simulink model "DIY_simuling"  (R2019a)
settings: Solver=ode23t  StartTime=0.0  StopTime=10  MaxStep=0.2  RelTol=1e-3
model workspace: external: MATLAB File D:\Users\bahaa\Desktop\gra_project\MATLAB\Assem1_DataFile.m (data not in the file)
undefined symbols (not defined in the file): ARM, J2, J3, J4, LEFT, RIGHT, Robot, smiData, TOP, X, Y, Z
libraries: sm_lib x92, nesl_utility x19
(part 1 of 3)
settings Model: Creator=bahaa  LastModifiedBy=bahaa

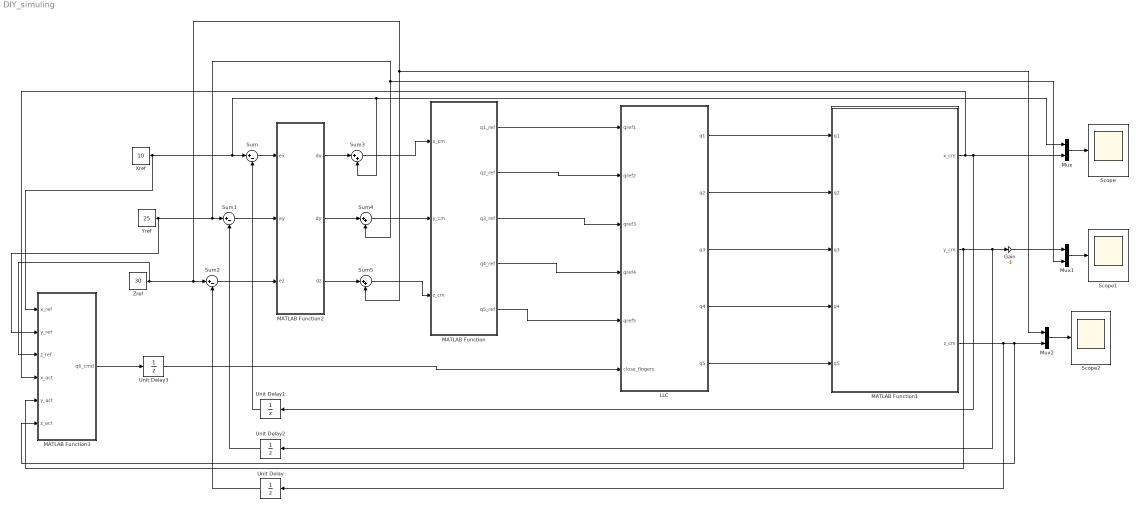
== system DIY_simuling ==
  Gain : Gain  Gain=-1
  LLC : Subsystem
  MATLAB Function : MATLAB Function  TreatAsAtomicUnit=on
  MATLAB Function1 : MATLAB Function  TreatAsAtomicUnit=on
  MATLAB Function2 : MATLAB Function  TreatAsAtomicUnit=on
  MATLAB Function3 : MATLAB Function  TreatAsAtomicUnit=on
  Mux : Mux  Inputs=2
  Mux1 : Mux  Inputs=2
  Mux2 : Mux  Inputs=2
  Scope : Scope
  Scope1 : Scope
  Scope2 : Scope
  Sum : Sum  Inputs=|+-
  Sum1 : Sum  Inputs=|+-
  Sum2 : Sum  Inputs=|+-
  Sum3 : Sum  Inputs=|++
  Sum4 : Sum  Inputs=|++
  Sum5 : Sum  Inputs=|++
  Unit Delay{,1..3} (4 alike) : UnitDelay  SampleTime=-1  HasFrameUpgradeWarning=on
  Xref : Constant  Value=10
  Yref : Constant  Value=25
  Zref : Constant  Value=30
  wires:
  Xref/1 -> MATLAB Function3/1(x_ref), Mux/1, Sum3/2, Sum/1
  Zref/1 -> MATLAB Function3/3(z_ref), Sum2/1, Sum5/2, Mux2/1
  Sum/1 -> MATLAB Function2/1(ex)
  Sum1/1 -> MATLAB Function2/2(ey)
  Sum2/1 -> MATLAB Function2/3(ez)
  MATLAB Function/1(q1_ref) -> LLC/1(qref1)
  MATLAB Function/2(q2_ref) -> LLC/2(qref2)
  MATLAB Function/3(q3_ref) -> LLC/3(qref3)
  MATLAB Function/4(q4_ref) -> LLC/4(qref4)
  MATLAB Function/5(q5_ref) -> LLC/5(qref5)
  LLC/1(q1) -> MATLAB Function1/1(q1)
  LLC/2(q2) -> MATLAB Function1/2(q2)
  LLC/3(q3) -> MATLAB Function1/3(q3)
  LLC/4(q4) -> MATLAB Function1/4(q4)
  LLC/5(q5) -> MATLAB Function1/5(q5)
  MATLAB Function1/2(y_cm) -> MATLAB Function3/5(y_act), Unit Delay2/1, Gain/1
  MATLAB Function1/3(z_cm) -> MATLAB Function3/6(z_act), Mux2/2, Unit Delay/1
  Mux/1 -> Scope/1
  Mux1/1 -> Scope1/1
  Mux2/1 -> Scope2/1
  MATLAB Function2/1(dx) -> Sum3/1
  MATLAB Function2/2(dy) -> Sum4/1
  MATLAB Function2/3(dz) -> Sum5/1
  Sum3/1 -> MATLAB Function/1(x_cm)
  Sum4/1 -> MATLAB Function/2(y_cm)
  Sum5/1 -> MATLAB Function/3(z_cm)
  Unit Delay/1 -> Sum2/2
  Unit Delay1/1 -> Sum/2
  Unit Delay2/1 -> Sum1/2
  MATLAB Function1/1(x_cm) -> MATLAB Function3/4(x_act), Mux/2, Unit Delay1/1
  MATLAB Function3/1(q6_cmd) -> Unit Delay3/1
  Unit Delay3/1 -> LLC/6(close_fingers)
  Yref/1 -> MATLAB Function3/2(y_ref), Mux1/2, Sum4/2, Sum1/1
  Gain/1 -> Mux1/1

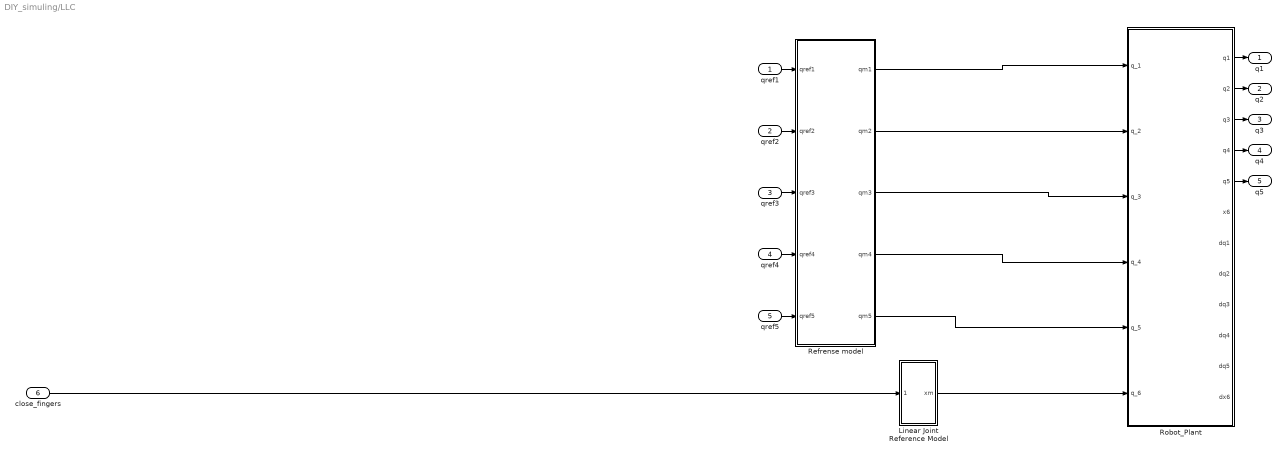
== system DIY_simuling/LLC ==
  qref1 : Inport
  qref2 : Inport  Port=2
  qref3 : Inport  Port=3
  qref4 : Inport  Port=4
  qref5 : Inport  Port=5
  close_fingers : Inport  Port=6
  Linear Joint Reference Model : Subsystem
  Refrense model : Subsystem
  Robot_Plant : Subsystem
  q1 : Outport
  q2 : Outport  Port=2
  q3 : Outport  Port=3
  q4 : Outport  Port=4
  q5 : Outport  Port=5
  wires:
  qref1/1 -> Refrense model/1(qref1)
  Refrense model/4(qm4) -> Robot_Plant/4(q_4)
  Refrense model/3(qm3) -> Robot_Plant/3(q_3)
  Linear Joint Reference Model/1(xm) -> Robot_Plant/6(q_6)
  Refrense model/1(qm1) -> Robot_Plant/1(q_1)
  Refrense model/2(qm2) -> Robot_Plant/2(q_2)
  Refrense model/5(qm5) -> Robot_Plant/5(q_5)
  Robot_Plant/1(q1) -> q1/1
  qref2/1 -> Refrense model/2(qref2)
  qref4/1 -> Refrense model/4(qref4)
  qref3/1 -> Refrense model/3(qref3)
  qref5/1 -> Refrense model/5(qref5)
  Robot_Plant/4(q4) -> q4/1
  Robot_Plant/3(q3) -> q3/1
  Robot_Plant/2(q2) -> q2/1
  Robot_Plant/5(q5) -> q5/1
  close_fingers/1 -> Linear Joint Reference Model/1(x6ref)

== system DIY_simuling/LLC/Linear Joint Reference Model ==
  x6ref : Inport
  Integrator : Integrator  InitialCondition=[0;0]
  MATLAB Function : MATLAB Function  TreatAsAtomicUnit=on
  xm : Outport
  wires:
  Integrator/1 -> MATLAB Function/2(xm6)
  MATLAB Function/1(xm6dot) -> Integrator/1
  MATLAB Function/2(x6_m) -> xm/1
  x6ref/1 -> MATLAB Function/1(x6_ref)

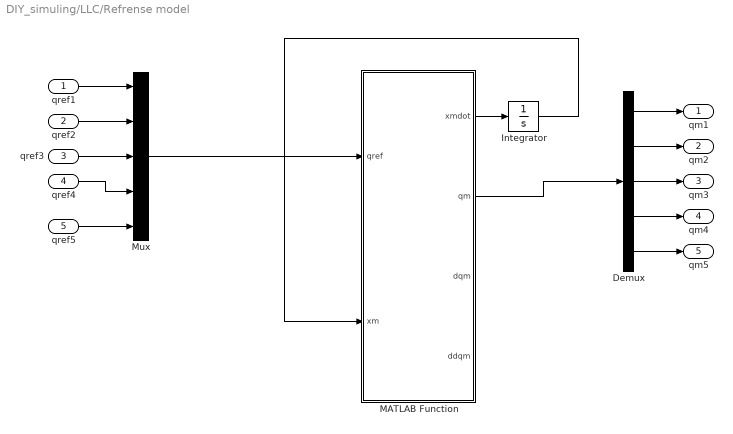
== system DIY_simuling/LLC/Refrense model ==
  qref1 : Inport
  qref2 : Inport  Port=2
  qref3 : Inport  Port=3
  qref4 : Inport  Port=4
  qref5 : Inport  Port=5
  Demux : Demux  Outputs=5
  Integrator : Integrator  InitialCondition=zeros(10,1)
  MATLAB Function : MATLAB Function  TreatAsAtomicUnit=on
  Mux : Mux  Inputs=5
  qm1 : Outport
  qm2 : Outport  Port=2
  qm3 : Outport  Port=3
  qm4 : Outport  Port=4
  qm5 : Outport  Port=5
  wires:
  MATLAB Function/1(xmdot) -> Integrator/1
  MATLAB Function/2(qm) -> Demux/1
  Integrator/1 -> MATLAB Function/2(xm)
  Demux/5 -> qm5/1
  Demux/4 -> qm4/1
  Demux/3 -> qm3/1
  Demux/2 -> qm2/1
  Demux/1 -> qm1/1
  qref1/1 -> Mux/1
  Mux/1 -> MATLAB Function/1(qref)
  qref2/1 -> Mux/2
  qref3/1 -> Mux/3
  qref4/1 -> Mux/4
  qref5/1 -> Mux/5

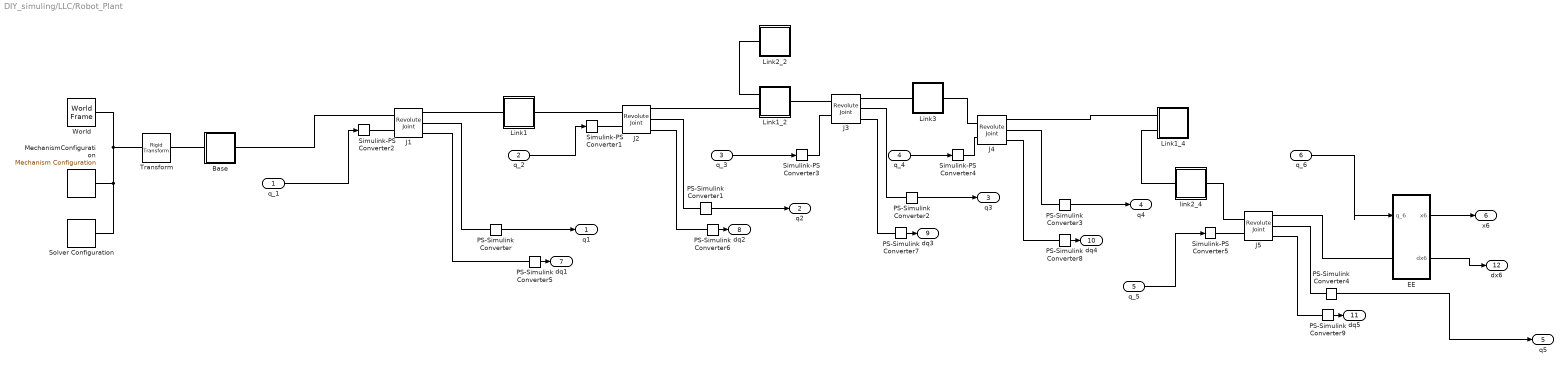
== system DIY_simuling/LLC/Robot_Plant ==
  q_1 : Inport
  q_2 : Inport  Port=2
  q_3 : Inport  Port=3
  q_4 : Inport  Port=4
  q_5 : Inport  Port=5
  q_6 : Inport  Port=6
  Base : Subsystem
  EE : Subsystem
  J1 : sm_lib/Joints/Revolute Joint  SenseConstraintForce=off  SenseConstraintForceX=off  SenseConstraintForceY=off  SenseConstraintForceZ=off  SenseConstraintTorque=off  SenseConstraintTorqueX=off  SenseConstraintTorqueY=off  SenseConstraintTorqueZ=off  SenseTotalForce=off  SenseTotalForceX=off  SenseTotalForceY=off  SenseTotalForceZ=off  SenseTotalTorque=off  SenseTotalTorqueX=off  SenseTotalTorqueY=off  SenseTotalTorqueZ=off  CompositeWrenchDir=FollowerOnBase  CompositeWrenchFrame=BaseFrame  EquilibriumPosition=0  EquilibriumPositionUnits=rad  SpringStiffness=0  SpringStiffnessUnits=N*m/rad  DampingCoefficient=0  DampingCoefficientUnits=N*m/(rad/s)  TorqueActuationMode=ComputedTorque  MotionActuationMode=InputMotion  SensePosition=on  SenseVelocity=on  SenseAcceleration=off  SenseTorqueForce=off  SenseLowerLimitTorqueForce=off  SenseUpperLimitTorqueForce=off  LowerLimitSpecify=on  LowerLimitBound=-90  LowerLimitBoundUnits=deg  LowerLimitStiffness=1e4  LowerLimitStiffnessUnits=N*m/deg  LowerLimitDamping=10  LowerLimitDampingUnits=N*m/(deg/s)  LowerLimitTransitionRegionWidth=0.1  LowerLimitTransitionRegionWidthUnits=deg  UpperLimitSpecify=on  UpperLimitBound=90  UpperLimitBoundUnits=deg  UpperLimitStiffness=1e4  UpperLimitStiffnessUnits=N*m/deg  UpperLimitDamping=10  UpperLimitDampingUnits=N*m/(deg/s)  UpperLimitTransitionRegionWidth=0.1  UpperLimitTransitionRegionWidthUnits=deg  PositionTargetSpecify=on  PositionTargetPriority=Low  PositionTargetValue=smiData.RevoluteJoint(5).Rz.Pos  PositionTargetValueUnits=deg  VelocityTargetSpecify=off  VelocityTargetPriority=High  VelocityTargetValue=0  VelocityTargetValueUnits=deg/s
  J2 : sm_lib/Joints/Revolute Joint  SenseConstraintForce=off  SenseConstraintForceX=off  SenseConstraintForceY=off  SenseConstraintForceZ=off  SenseConstraintTorque=off  SenseConstraintTorqueX=off  SenseConstraintTorqueY=off  SenseConstraintTorqueZ=off  SenseTotalForce=off  SenseTotalForceX=off  SenseTotalForceY=off  SenseTotalForceZ=off  SenseTotalTorque=off  SenseTotalTorqueX=off  SenseTotalTorqueY=off  SenseTotalTorqueZ=off  CompositeWrenchDir=FollowerOnBase  CompositeWrenchFrame=BaseFrame  EquilibriumPosition=0  EquilibriumPositionUnits=rad  SpringStiffness=0  SpringStiffnessUnits=N*m/rad  DampingCoefficient=0  DampingCoefficientUnits=N*m/(rad/s)  TorqueActuationMode=ComputedTorque  MotionActuationMode=InputMotion  SensePosition=on  SenseVelocity=on  SenseAcceleration=off  SenseTorqueForce=off  SenseLowerLimitTorqueForce=off  SenseUpperLimitTorqueForce=off  LowerLimitSpecify=on  LowerLimitBound=-90  LowerLimitBoundUnits=deg  LowerLimitStiffness=1e4  LowerLimitStiffnessUnits=N*m/deg  LowerLimitDamping=10  LowerLimitDampingUnits=N*m/(deg/s)  LowerLimitTransitionRegionWidth=0.1  LowerLimitTransitionRegionWidthUnits=deg  UpperLimitSpecify=on  UpperLimitBound=90  UpperLimitBoundUnits=deg  UpperLimitStiffness=1e4  UpperLimitStiffnessUnits=N*m/deg  UpperLimitDamping=10  UpperLimitDampingUnits=N*m/(deg/s)  UpperLimitTransitionRegionWidth=0.1  UpperLimitTransitionRegionWidthUnits=deg  PositionTargetSpecify=on  PositionTargetPriority=Low  PositionTargetValue=smiData.RevoluteJoint(6).Rz.Pos  PositionTargetValueUnits=deg  VelocityTargetSpecify=off  VelocityTargetPriority=High  VelocityTargetValue=0  VelocityTargetValueUnits=deg/s
  J3 : sm_lib/Joints/Revolute Joint  SenseConstraintForce=off  SenseConstraintForceX=off  SenseConstraintForceY=off  SenseConstraintForceZ=off  SenseConstraintTorque=off  SenseConstraintTorqueX=off  SenseConstraintTorqueY=off  SenseConstraintTorqueZ=off  SenseTotalForce=off  SenseTotalForceX=off  SenseTotalForceY=off  SenseTotalForceZ=off  SenseTotalTorque=off  SenseTotalTorqueX=off  SenseTotalTorqueY=off  SenseTotalTorqueZ=off  CompositeWrenchDir=FollowerOnBase  CompositeWrenchFrame=BaseFrame  EquilibriumPosition=0  EquilibriumPositionUnits=rad  SpringStiffness=0  SpringStiffnessUnits=N*m/rad  DampingCoefficient=0  DampingCoefficientUnits=N*m/(rad/s)  TorqueActuationMode=ComputedTorque  MotionActuationMode=InputMotion  SensePosition=on  SenseVelocity=on  SenseAcceleration=off  SenseTorqueForce=off  SenseLowerLimitTorqueForce=off  SenseUpperLimitTorqueForce=off  LowerLimitSpecify=on  LowerLimitBound=-90  LowerLimitBoundUnits=deg  LowerLimitStiffness=1e4  LowerLimitStiffnessUnits=N*m/deg  LowerLimitDamping=10  LowerLimitDampingUnits=N*m/(deg/s)  LowerLimitTransitionRegionWidth=0.1  LowerLimitTransitionRegionWidthUnits=deg  UpperLimitSpecify=on  UpperLimitBound=90  UpperLimitBoundUnits=deg  UpperLimitStiffness=1e4  UpperLimitStiffnessUnits=N*m/deg  UpperLimitDamping=10  UpperLimitDampingUnits=N*m/(deg/s)  UpperLimitTransitionRegionWidth=0.1  UpperLimitTransitionRegionWidthUnits=deg  PositionTargetSpecify=on  PositionTargetPriority=Low  PositionTargetValue=smiData.RevoluteJoint(13).Rz.Pos  PositionTargetValueUnits=deg  VelocityTargetSpecify=off  VelocityTargetPriority=High  VelocityTargetValue=0  VelocityTargetValueUnits=deg/s
  J4 : sm_lib/Joints/Revolute Joint  SenseConstraintForce=off  SenseConstraintForceX=off  SenseConstraintForceY=off  SenseConstraintForceZ=off  SenseConstraintTorque=off  SenseConstraintTorqueX=off  SenseConstraintTorqueY=off  SenseConstraintTorqueZ=off  SenseTotalForce=off  SenseTotalForceX=off  SenseTotalForceY=off  SenseTotalForceZ=off  SenseTotalTorque=off  SenseTotalTorqueX=off  SenseTotalTorqueY=off  SenseTotalTorqueZ=off  CompositeWrenchDir=FollowerOnBase  CompositeWrenchFrame=BaseFrame  EquilibriumPosition=0  EquilibriumPositionUnits=rad  SpringStiffness=0  SpringStiffnessUnits=N*m/rad  DampingCoefficient=0  DampingCoefficientUnits=N*m/(rad/s)  TorqueActuationMode=ComputedTorque  MotionActuationMode=InputMotion  SensePosition=on  SenseVelocity=on  SenseAcceleration=off  SenseTorqueForce=off  SenseLowerLimitTorqueForce=off  SenseUpperLimitTorqueForce=off  LowerLimitSpecify=on  LowerLimitBound=-90  LowerLimitBoundUnits=deg  LowerLimitStiffness=1e4  LowerLimitStiffnessUnits=N*m/deg  LowerLimitDamping=10  LowerLimitDampingUnits=N*m/(deg/s)  LowerLimitTransitionRegionWidth=0.1  LowerLimitTransitionRegionWidthUnits=deg  UpperLimitSpecify=on  UpperLimitBound=90  UpperLimitBoundUnits=deg  UpperLimitStiffness=1e4  UpperLimitStiffnessUnits=N*m/deg  UpperLimitDamping=10  UpperLimitDampingUnits=N*m/(deg/s)  UpperLimitTransitionRegionWidth=0.1  UpperLimitTransitionRegionWidthUnits=deg  PositionTargetSpecify=on  PositionTargetPriority=Low  PositionTargetValue=smiData.RevoluteJoint(14).Rz.Pos  PositionTargetValueUnits=deg  VelocityTargetSpecify=off  VelocityTargetPriority=High  VelocityTargetValue=0  VelocityTargetValueUnits=deg/s
  J5 : sm_lib/Joints/Revolute Joint  SenseConstraintForce=off  SenseConstraintForceX=off  SenseConstraintForceY=off  SenseConstraintForceZ=off  SenseConstraintTorque=off  SenseConstraintTorqueX=off  SenseConstraintTorqueY=off  SenseConstraintTorqueZ=off  SenseTotalForce=off  SenseTotalForceX=off  SenseTotalForceY=off  SenseTotalForceZ=off  SenseTotalTorque=off  SenseTotalTorqueX=off  SenseTotalTorqueY=off  SenseTotalTorqueZ=off  CompositeWrenchDir=FollowerOnBase  CompositeWrenchFrame=BaseFrame  EquilibriumPosition=0  EquilibriumPositionUnits=rad  SpringStiffness=0  SpringStiffnessUnits=N*m/rad  DampingCoefficient=0  DampingCoefficientUnits=N*m/(rad/s)  TorqueActuationMode=ComputedTorque  MotionActuationMode=InputMotion  SensePosition=on  SenseVelocity=on  SenseAcceleration=off  SenseTorqueForce=off  SenseLowerLimitTorqueForce=off  SenseUpperLimitTorqueForce=off  LowerLimitSpecify=on  LowerLimitBound=-90  LowerLimitBoundUnits=deg  LowerLimitStiffness=1e4  LowerLimitStiffnessUnits=N*m/deg  LowerLimitDamping=10  LowerLimitDampingUnits=N*m/(deg/s)  LowerLimitTransitionRegionWidth=0.1  LowerLimitTransitionRegionWidthUnits=deg  UpperLimitSpecify=on  UpperLimitBound=90  UpperLimitBoundUnits=deg  UpperLimitStiffness=1e4  UpperLimitStiffnessUnits=N*m/deg  UpperLimitDamping=10  UpperLimitDampingUnits=N*m/(deg/s)  UpperLimitTransitionRegionWidth=0.1  UpperLimitTransitionRegionWidthUnits=deg  PositionTargetSpecify=on  PositionTargetPriority=Low  PositionTargetValue=smiData.RevoluteJoint(4).Rz.Pos  PositionTargetValueUnits=deg  VelocityTargetSpecify=off  VelocityTargetPriority=High  VelocityTargetValue=0  VelocityTargetValueUnits=deg/s
  Link1 : Subsystem
  Link1_2 : Subsystem
  Link1_4 : Subsystem
  Link2_2 : Subsystem
  Link3 : Subsystem
  MechanismConfiguration : sm_lib/Utilities/Mechanism Configuration  UniformGravity=Constant  GravityVector=[0 -9.80665 0]  GravityUnits=m/s^2  LinearizationDelta=0.001
  PS-Simulink Converter{,1..4} (5 alike) : nesl_utility/PS-Simulink Converter  PhysicalDomain=network_engine_domain  SubClassName=ps_output  LeftPortType=input  RightPortType=output  PseudoPeriodic=off  Frequencies=[]  Unit=rad  AffineConversion=off
  PS-Simulink Converter{5..9} (5 alike) : nesl_utility/PS-Simulink Converter  PhysicalDomain=network_engine_domain  SubClassName=ps_output  LeftPortType=input  RightPortType=output  PseudoPeriodic=off  Frequencies=[]  Unit=rad/s  AffineConversion=off
  Simulink-PS Converter{1..5} (5 alike) : nesl_utility/Simulink-PS Converter  PhysicalDomain=network_engine_domain  SubClassName=ps_input  LeftPortType=input  RightPortType=output  PseudoPeriodic=off  Frequencies=[]  NoiseDistribution=none  NoiseParameters=[]  Unit=rad  AffineConversion=off  FilteringAndDerivatives=filter  SimscapeFilterOrder=2  InputFilterTimeConstant=0.001  UdotUserProvided=0
  Solver Configuration : nesl_utility/Solver Configuration  PhysicalDomain=network_engine_domain  SubClassName=solver  LeftPortType=input  RightPortType=generic  Tones=[]  Harmonics=[]  SimulateNoise=off  Profile=off  UseLocalSampling=off  EnableSwitchedLinearOptims=on  FrequencyDomain=off  UseCCode=off  RelTol=0.001  AbsTol=1e-06  MinStep=1e-09  ToWorkspace=off  RevertToSquareIcSolve=off  NumHomotopyIterations=100  PhasorMode=off  PhasorModeNumHarmonics=1  DoDC=off  ResidualTolerance=1e-09  UseLocalSolver=off  LocalSolverChoice=NE_BACKWARD_EULER_ADVANCER  LocalSolverSampleTime=0.001  DoFixedCost=off  MaxNonlinIter=3  MaxModeIter=2  LinearAlgebra=auto  EquationFormulation=NE_TIME_EF  DelaysMemoryBudget=1024  AutomaticFiltering=on  FilteringTimeConstant=0.001  PartitionStorageMethod=AS_NEEDED  PartitionMemoryBudget=1024  PartitionMethod=ROBUST
  Transform : sm_lib/Frames and Transforms/Rigid Transform  TranslationMethod=Cartesian  TranslationStandardOffset=0  TranslationLengthUnit=mm  TranslationStandardAxis=+Z  TranslationCartesianOffset=smiData.RigidTransform(39).translation  TranslationROffset=0  TranslationROffsetUnits=m  TranslationZOffset=0  TranslationZOffsetUnits=m  TranslationThetaOffset=0  TranslationThetaOffsetUnits=deg  RotationMethod=RotationSequence  RotationAngleUnits=rad  RotationStandardAxis=+Z  RotationAngle=smiData.RigidTransform(39).angle  RotationArbitraryAxis=smiData.RigidTransform(39).axis  FollAlignAxisA=+X  BaseAlignAxisA=+Y  FollAlignAxisB=+Y  BaseAlignAxisB=+Z  RotationSequenceAxes=BaseAxes  RotationSequence=XYZ  RotationSequenceAngles="[90  0 90]"  RotationSequenceAnglesUnits=deg  RotationMatrix=[1 0 0; 0 1 0; 0 0 1]
  World : sm_lib/Frames and Transforms/World Frame
  link2_4 : Subsystem
  q1 : Outport
  q2 : Outport  Port=2
  q3 : Outport  Port=3
  q4 : Outport  Port=4
  q5 : Outport  Port=5
  x6 : Outport  Port=6
  dq1 : Outport  Port=7
  dq2 : Outport  Port=8
  dq3 : Outport  Port=9
  dq4 : Outport  Port=10
  dq5 : Outport  Port=11
  dx6 : Outport  Port=12
  wires:
  q_6/1 -> EE/1(q_6)
  EE/1(x6) -> x6/1
  PS-Simulink Converter5/1 -> dq1/1
  PS-Simulink Converter6/1 -> dq2/1
  PS-Simulink Converter7/1 -> dq3/1
  PS-Simulink Converter8/1 -> dq4/1
  PS-Simulink Converter9/1 -> dq5/1
  EE/2(dx6) -> dx6/1
  q_1/1 -> Simulink-PS Converter2/1
  q_2/1 -> Simulink-PS Converter1/1
  q_3/1 -> Simulink-PS Converter3/1
  q_4/1 -> Simulink-PS Converter4/1
  q_5/1 -> Simulink-PS Converter5/1
  PS-Simulink Converter/1 -> q1/1
  PS-Simulink Converter1/1 -> q2/1
  PS-Simulink Converter2/1 -> q3/1
  PS-Simulink Converter3/1 -> q4/1
  PS-Simulink Converter4/1 -> q5/1
  connections:
  Link1_4/LConn2 -- link2_4/LConn1
  J2/RConn1 -- Link1_2/LConn2
  J4/RConn1 -- Link1_4/LConn1
  PS-Simulink Converter1/LConn1 -- J2/RConn2
  J4/LConn1 -- Link3/RConn1
  Transform/LConn1 -- MechanismConfiguration/RConn1 -- Solver Configuration/RConn1 -- World/RConn1
  PS-Simulink Converter2/LConn1 -- J3/RConn2
  J5/RConn1 -- EE/LConn1
  Simulink-PS Converter4/RConn1 -- J4/LConn2
  PS-Simulink Converter/LConn1 -- J1/RConn2
  PS-Simulink Converter4/LConn1 -- J5/RConn2
  J1/RConn1 -- Link1/LConn1
  Simulink-PS Converter2/RConn1 -- J1/LConn2
  Link1_2/LConn1 -- Link2_2/LConn1
  J3/LConn1 -- Link1_2/RConn1
  J3/RConn1 -- Link3/LConn1
  Simulink-PS Converter1/RConn1 -- J2/LConn2
  Simulink-PS Converter3/RConn1 -- J3/LConn2
  PS-Simulink Converter3/LConn1 -- J4/RConn2
  J2/LConn1 -- Link1/RConn1
  J1/LConn1 -- Base/RConn1
  Base/LConn1 -- Transform/RConn1
  J5/LConn1 -- link2_4/RConn1
  Simulink-PS Converter5/RConn1 -- J5/LConn2
  J1/RConn3 -- PS-Simulink Converter5/LConn1
  PS-Simulink Converter6/LConn1 -- J2/RConn3
  PS-Simulink Converter7/LConn1 -- J3/RConn3
  PS-Simulink Converter8/LConn1 -- J4/RConn3
  J5/RConn3 -- PS-Simulink Converter9/LConn1

== system DIY_simuling/LLC/Robot_Plant/Base ==
  ReferenceFrame : sm_lib/Frames and Transforms/Reference Frame
  Solid : sm_lib/Body Elements/Solid  InertiaType=Custom  Mass=smiData.Solid(1).mass  MassUnits=kg  CenterOfMass=smiData.Solid(1).CoM  CenterOfMassUnits=mm  MomentsOfInertia=smiData.Solid(1).MoI  MomentsOfInertiaUnits=kg*mm^2  ProductsOfInertia=smiData.Solid(1).PoI  ProductsOfInertiaUnits=kg*mm^2  BasedOnType=Density  Density=1000  DensityUnits=kg/m^3  DoExposeReferenceFrame=on  SerializedFrames=<Frames/>  GraphicType=FromGeometry  MarkerShape=Sphere  MarkerSize=10  GraphicVisPropType=SimpleVisualProperties  GraphicDiffuseColor=smiData.Solid(1).color  GraphicSpecularColor=[0.5 0.5 0.5 1.0]  GraphicAmbientColor=[0.15 0.15 0.15 1.0]  GraphicEmissiveColor=[0.0 0.0 0.0 1.0]  GraphicShininess=75  GraphicOpacity=smiData.Solid(1).opacity  GeometryShape=FromFile  RectangleSize=[1 1]  RectangleSizeUnits=m  BrickDimensions=[1 1 1]  BrickDimensionUnits=m  CylinderRadius=1  CylinderRadiusUnits=m  CylinderLength=1  CylinderLengthUnits=m  SphereRadius=1  SphereRadiusUnits=m  EllipsoidRadii=[1 1 1]  EllipsoidRadiiUnits=m  ExtrusionCrossSection=[1 1; -1 1; -1 -1; 1 -1]  ExtrusionCrossSectionUnits=m  ExtrusionLength=1  ExtrusionLengthUnits=m  PolygonNumSides=3  PolygonOuterRadius=1  PolygonOuterRadiusUnits=m  ExtGeomFileType=STEP  ExtGeomFileName=Robot - Base.step_Default_sldprt.STEP  ExtGeomFileUnits=m  RevolutionCrossSection=[1 1; 1 -1; 2 -1; 2 1]  RevolutionCrossSectionUnits=m  RevolutionExtent=Full  RevolutionAngle=180  RevolutionAngleUnits=deg
  Transform : sm_lib/Frames and Transforms/Rigid Transform  TranslationMethod=Cartesian  TranslationStandardOffset=0  TranslationLengthUnit=mm  TranslationStandardAxis=+Z  TranslationCartesianOffset=smiData.RigidTransform(9).translation  TranslationROffset=0  TranslationROffsetUnits=m  TranslationZOffset=0  TranslationZOffsetUnits=m  TranslationThetaOffset=0  TranslationThetaOffsetUnits=deg  RotationMethod=ArbitraryAxis  RotationAngleUnits=rad  RotationStandardAxis=+Z  RotationAngle=smiData.RigidTransform(9).angle  RotationArbitraryAxis=smiData.RigidTransform(9).axis  FollAlignAxisA=+X  BaseAlignAxisA=+Y  FollAlignAxisB=+Y  BaseAlignAxisB=+Z  RotationSequenceAxes=FollowerAxes  RotationSequence=XYX  RotationSequenceAngles=[0 0 0]  RotationSequenceAnglesUnits=deg  RotationMatrix=[1 0 0; 0 1 0; 0 0 1]
  F1 : PMIOPort  Side=Left
  F : PMIOPort  Port=2  Side=Right
  connections:
  Solid/RConn1 -- ReferenceFrame/RConn1 -- Transform/LConn1 -- F1/RConn1
  Transform/RConn1 -- F/RConn1

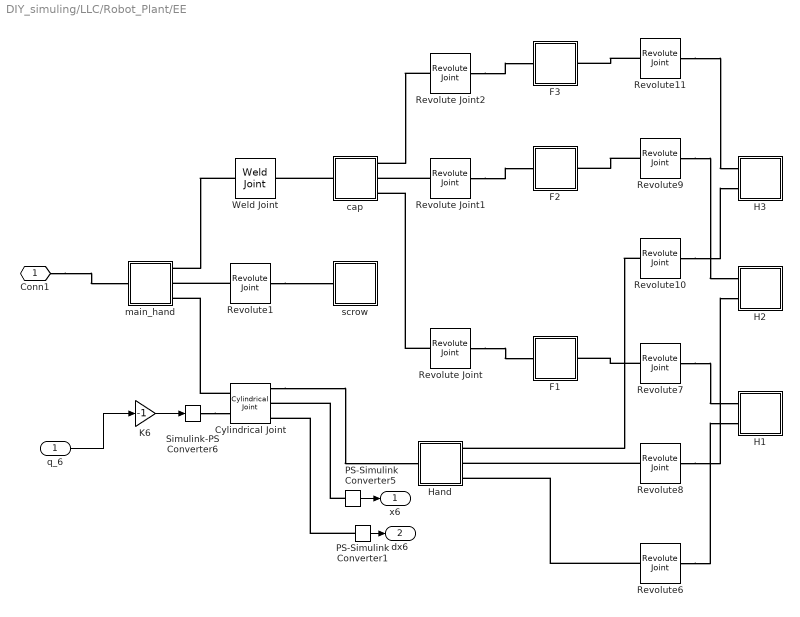
== system DIY_simuling/LLC/Robot_Plant/EE ==
  q_6 : Inport
  Cylindrical Joint : sm_lib/Joints/Cylindrical Joint  SenseConstraintForce=off  SenseConstraintForceX=off  SenseConstraintForceY=off  SenseConstraintForceZ=off  SenseConstraintTorque=off  SenseConstraintTorqueX=off  SenseConstraintTorqueY=off  SenseConstraintTorqueZ=off  SenseTotalForce=off  SenseTotalForceX=off  SenseTotalForceY=off  SenseTotalForceZ=off  SenseTotalTorque=off  SenseTotalTorqueX=off  SenseTotalTorqueY=off  SenseTotalTorqueZ=off  CompositeWrenchDir=FollowerOnBase  CompositeWrenchFrame=BaseFrame  PzEquilibriumPosition=0  PzEquilibriumPositionUnits=m  PzSpringStiffness=0  PzSpringStiffnessUnits=N/m  PzDampingCoefficient=0  PzDampingCoefficientUnits=N/(m/s)  PzTorqueActuationMode=ComputedTorque  PzMotionActuationMode=InputMotion  PzSensePosition=on  PzSenseVelocity=on  PzSenseAcceleration=off  PzSenseTorqueForce=off  PzSenseLowerLimitTorqueForce=off  PzSenseUpperLimitTorqueForce=off  PzLowerLimitSpecify=on  PzLowerLimitBound=0  PzLowerLimitBoundUnits=m  PzLowerLimitStiffness=1e6  PzLowerLimitStiffnessUnits=N/m  PzLowerLimitDamping=1e3  PzLowerLimitDampingUnits=N/(m/s)  PzLowerLimitTransitionRegionWidth=1e-4  PzLowerLimitTransitionRegionWidthUnits=m  PzUpperLimitSpecify=on  PzUpperLimitBound=0.022  PzUpperLimitBoundUnits=m  PzUpperLimitStiffness=1e6  PzUpperLimitStiffnessUnits=N/m  PzUpperLimitDamping=1e3  PzUpperLimitDampingUnits=N/(m/s)  PzUpperLimitTransitionRegionWidth=1e-4  PzUpperLimitTransitionRegionWidthUnits=m  PzPositionTargetSpecify=off  PzPositionTargetPriority=High  PzPositionTargetValue=0  PzPositionTargetValueUnits=m  PzVelocityTargetSpecify=off  PzVelocityTargetPriority=High  PzVelocityTargetValue=0  PzVelocityTargetValueUnits=m/s  RzEquilibriumPosition=0  RzEquilibriumPositionUnits=deg  RzSpringStiffness=0  RzSpringStiffnessUnits=N*m/deg  RzDampingCoefficient=0  RzDampingCoefficientUnits=N*m/(deg/s)  RzTorqueActuationMode=NoTorque  RzMotionActuationMode=ComputedMotion  RzSensePosition=off  RzSenseVelocity=off  RzSenseAcceleration=off  RzSenseTorqueForce=off  RzSenseLowerLimitTorqueForce=off  RzSenseUpperLimitTorqueForce=off  RzLowerLimitSpecify=on  RzLowerLimitBound=-1  RzLowerLimitBoundUnits=deg  RzLowerLimitStiffness=1e4  RzLowerLimitStiffnessUnits=N*m/deg  RzLowerLimitDamping=10  RzLowerLimitDampingUnits=N*m/(deg/s)  RzLowerLimitTransitionRegionWidth=0.1  RzLowerLimitTransitionRegionWidthUnits=deg  RzUpperLimitSpecify=on  RzUpperLimitBound=1  RzUpperLimitBoundUnits=deg  RzUpperLimitStiffness=1e4  RzUpperLimitStiffnessUnits=N*m/deg  RzUpperLimitDamping=10  RzUpperLimitDampingUnits=N*m/(deg/s)  RzUpperLimitTransitionRegionWidth=0.1  RzUpperLimitTransitionRegionWidthUnits=deg  RzPositionTargetSpecify=off  RzPositionTargetPriority=High  RzPositionTargetValue=0  RzPositionTargetValueUnits=deg  RzVelocityTargetSpecify=off  RzVelocityTargetPriority=High  RzVelocityTargetValue=0  RzVelocityTargetValueUnits=deg/s
  F1 : Subsystem
  F2 : Subsystem
  F3 : Subsystem
  H1 : Subsystem
  H2 : Subsystem
  H3 : Subsystem
  Hand : Subsystem
  K6 : Gain  Gain=-1
  PS-Simulink Converter1 : nesl_utility/PS-Simulink Converter  PhysicalDomain=network_engine_domain  SubClassName=ps_output  LeftPortType=input  RightPortType=output  PseudoPeriodic=off  Frequencies=[]  Unit=m/s  AffineConversion=off
  PS-Simulink Converter5 : nesl_utility/PS-Simulink Converter  PhysicalDomain=network_engine_domain  SubClassName=ps_output  LeftPortType=input  RightPortType=output  PseudoPeriodic=off  Frequencies=[]  Unit=m  AffineConversion=off
  Revolute Joint : sm_lib/Joints/Revolute Joint  SenseConstraintForce=off  SenseConstraintForceX=off  SenseConstraintForceY=off  SenseConstraintForceZ=off  SenseConstraintTorque=off  SenseConstraintTorqueX=off  SenseConstraintTorqueY=off  SenseConstraintTorqueZ=off  SenseTotalForce=off  SenseTotalForceX=off  SenseTotalForceY=off  SenseTotalForceZ=off  SenseTotalTorque=off  SenseTotalTorqueX=off  SenseTotalTorqueY=off  SenseTotalTorqueZ=off  CompositeWrenchDir=FollowerOnBase  CompositeWrenchFrame=BaseFrame  EquilibriumPosition=0  EquilibriumPositionUnits=deg  SpringStiffness=0  SpringStiffnessUnits=N*m/deg  DampingCoefficient=0  DampingCoefficientUnits=N*m/(deg/s)  TorqueActuationMode=NoTorque  MotionActuationMode=ComputedMotion  SensePosition=off  SenseVelocity=off  SenseAcceleration=off  SenseTorqueForce=off  SenseLowerLimitTorqueForce=off  SenseUpperLimitTorqueForce=off  LowerLimitSpecify=off  LowerLimitBound=-90  LowerLimitBoundUnits=deg  LowerLimitStiffness=1e4  LowerLimitStiffnessUnits=N*m/deg  LowerLimitDamping=10  LowerLimitDampingUnits=N*m/(deg/s)  LowerLimitTransitionRegionWidth=0.1  LowerLimitTransitionRegionWidthUnits=deg  UpperLimitSpecify=off  UpperLimitBound=90  UpperLimitBoundUnits=deg  UpperLimitStiffness=1e4  UpperLimitStiffnessUnits=N*m/deg  UpperLimitDamping=10  UpperLimitDampingUnits=N*m/(deg/s)  UpperLimitTransitionRegionWidth=0.1  UpperLimitTransitionRegionWidthUnits=deg  PositionTargetSpecify=off  PositionTargetPriority=High  PositionTargetValue=0  PositionTargetValueUnits=deg  VelocityTargetSpecify=off  VelocityTargetPriority=High  VelocityTargetValue=0  VelocityTargetValueUnits=deg/s
  Revolute Joint1 : sm_lib/Joints/Revolute Joint  SenseConstraintForce=off  SenseConstraintForceX=off  SenseConstraintForceY=off  SenseConstraintForceZ=off  SenseConstraintTorque=off  SenseConstraintTorqueX=off  SenseConstraintTorqueY=off  SenseConstraintTorqueZ=off  SenseTotalForce=off  SenseTotalForceX=off  SenseTotalForceY=off  SenseTotalForceZ=off  SenseTotalTorque=off  SenseTotalTorqueX=off  SenseTotalTorqueY=off  SenseTotalTorqueZ=off  CompositeWrenchDir=FollowerOnBase  CompositeWrenchFrame=BaseFrame  EquilibriumPosition=0  EquilibriumPositionUnits=deg  SpringStiffness=0  SpringStiffnessUnits=N*m/deg  DampingCoefficient=0  DampingCoefficientUnits=N*m/(deg/s)  TorqueActuationMode=NoTorque  MotionActuationMode=ComputedMotion  SensePosition=off  SenseVelocity=off  SenseAcceleration=off  SenseTorqueForce=off  SenseLowerLimitTorqueForce=off  SenseUpperLimitTorqueForce=off  LowerLimitSpecify=off  LowerLimitBound=-90  LowerLimitBoundUnits=deg  LowerLimitStiffness=1e4  LowerLimitStiffnessUnits=N*m/deg  LowerLimitDamping=10  LowerLimitDampingUnits=N*m/(deg/s)  LowerLimitTransitionRegionWidth=0.1  LowerLimitTransitionRegionWidthUnits=deg  UpperLimitSpecify=off  UpperLimitBound=90  UpperLimitBoundUnits=deg  UpperLimitStiffness=1e4  UpperLimitStiffnessUnits=N*m/deg  UpperLimitDamping=10  UpperLimitDampingUnits=N*m/(deg/s)  UpperLimitTransitionRegionWidth=0.1  UpperLimitTransitionRegionWidthUnits=deg  PositionTargetSpecify=off  PositionTargetPriority=High  PositionTargetValue=0  PositionTargetValueUnits=deg  VelocityTargetSpecify=off  VelocityTargetPriority=High  VelocityTargetValue=0  VelocityTargetValueUnits=deg/s
  Revolute Joint2 : sm_lib/Joints/Revolute Joint  SenseConstraintForce=off  SenseConstraintForceX=off  SenseConstraintForceY=off  SenseConstraintForceZ=off  SenseConstraintTorque=off  SenseConstraintTorqueX=off  SenseConstraintTorqueY=off  SenseConstraintTorqueZ=off  SenseTotalForce=off  SenseTotalForceX=off  SenseTotalForceY=off  SenseTotalForceZ=off  SenseTotalTorque=off  SenseTotalTorqueX=off  SenseTotalTorqueY=off  SenseTotalTorqueZ=off  CompositeWrenchDir=FollowerOnBase  CompositeWrenchFrame=BaseFrame  EquilibriumPosition=0  EquilibriumPositionUnits=deg  SpringStiffness=0  SpringStiffnessUnits=N*m/deg  DampingCoefficient=0  DampingCoefficientUnits=N*m/(deg/s)  TorqueActuationMode=NoTorque  MotionActuationMode=ComputedMotion  SensePosition=off  SenseVelocity=off  SenseAcceleration=off  SenseTorqueForce=off  SenseLowerLimitTorqueForce=off  SenseUpperLimitTorqueForce=off  LowerLimitSpecify=off  LowerLimitBound=-90  LowerLimitBoundUnits=deg  LowerLimitStiffness=1e4  LowerLimitStiffnessUnits=N*m/deg  LowerLimitDamping=10  LowerLimitDampingUnits=N*m/(deg/s)  LowerLimitTransitionRegionWidth=0.1  LowerLimitTransitionRegionWidthUnits=deg  UpperLimitSpecify=off  UpperLimitBound=90  UpperLimitBoundUnits=deg  UpperLimitStiffness=1e4  UpperLimitStiffnessUnits=N*m/deg  UpperLimitDamping=10  UpperLimitDampingUnits=N*m/(deg/s)  UpperLimitTransitionRegionWidth=0.1  UpperLimitTransitionRegionWidthUnits=deg  PositionTargetSpecify=off  PositionTargetPriority=High  PositionTargetValue=0  PositionTargetValueUnits=deg  VelocityTargetSpecify=off  VelocityTargetPriority=High  VelocityTargetValue=0  VelocityTargetValueUnits=deg/s
  Revolute1 : sm_lib/Joints/Revolute Joint  SenseConstraintForce=off  SenseConstraintForceX=off  SenseConstraintForceY=off  SenseConstraintForceZ=off  SenseConstraintTorque=off  SenseConstraintTorqueX=off  SenseConstraintTorqueY=off  SenseConstraintTorqueZ=off  SenseTotalForce=off  SenseTotalForceX=off  SenseTotalForceY=off  SenseTotalForceZ=off  SenseTotalTorque=off  SenseTotalTorqueX=off  SenseTotalTorqueY=off  SenseTotalTorqueZ=off  CompositeWrenchDir=FollowerOnBase  CompositeWrenchFrame=BaseFrame  EquilibriumPosition=0  EquilibriumPositionUnits=rad  SpringStiffness=0  SpringStiffnessUnits=N*m/rad  DampingCoefficient=0  DampingCoefficientUnits=N*m/(rad/s)  TorqueActuationMode=NoTorque  MotionActuationMode=ComputedMotion  SensePosition=off  SenseVelocity=off  SenseAcceleration=off  SenseTorqueForce=off  SenseLowerLimitTorqueForce=off  SenseUpperLimitTorqueForce=off  LowerLimitSpecify=off  LowerLimitBound=-90  LowerLimitBoundUnits=deg  LowerLimitStiffness=1e4  LowerLimitStiffnessUnits=N*m/deg  LowerLimitDamping=10  LowerLimitDampingUnits=N*m/(deg/s)  LowerLimitTransitionRegionWidth=0.1  LowerLimitTransitionRegionWidthUnits=deg  UpperLimitSpecify=off  UpperLimitBound=90  UpperLimitBoundUnits=deg  UpperLimitStiffness=1e4  UpperLimitStiffnessUnits=N*m/deg  UpperLimitDamping=10  UpperLimitDampingUnits=N*m/(deg/s)  UpperLimitTransitionRegionWidth=0.1  UpperLimitTransitionRegionWidthUnits=deg  PositionTargetSpecify=on  PositionTargetPriority=Low  PositionTargetValue=smiData.RevoluteJoint(2).Rz.Pos  PositionTargetValueUnits=deg  VelocityTargetSpecify=off  VelocityTargetPriority=High  VelocityTargetValue=0  VelocityTargetValueUnits=deg/s
  Revolute10 : sm_lib/Joints/Revolute Joint  SenseConstraintForce=off  SenseConstraintForceX=off  SenseConstraintForceY=off  SenseConstraintForceZ=off  SenseConstraintTorque=off  SenseConstraintTorqueX=off  SenseConstraintTorqueY=off  SenseConstraintTorqueZ=off  SenseTotalForce=off  SenseTotalForceX=off  SenseTotalForceY=off  SenseTotalForceZ=off  SenseTotalTorque=off  SenseTotalTorqueX=off  SenseTotalTorqueY=off  SenseTotalTorqueZ=off  CompositeWrenchDir=FollowerOnBase  CompositeWrenchFrame=BaseFrame  EquilibriumPosition=0  EquilibriumPositionUnits=rad  SpringStiffness=0  SpringStiffnessUnits=N*m/rad  DampingCoefficient=0  DampingCoefficientUnits=N*m/(rad/s)  TorqueActuationMode=NoTorque  MotionActuationMode=ComputedMotion  SensePosition=off  SenseVelocity=off  SenseAcceleration=off  SenseTorqueForce=off  SenseLowerLimitTorqueForce=off  SenseUpperLimitTorqueForce=off  LowerLimitSpecify=off  LowerLimitBound=-90  LowerLimitBoundUnits=deg  LowerLimitStiffness=1e4  LowerLimitStiffnessUnits=N*m/deg  LowerLimitDamping=10  LowerLimitDampingUnits=N*m/(deg/s)  LowerLimitTransitionRegionWidth=0.1  LowerLimitTransitionRegionWidthUnits=deg  UpperLimitSpecify=off  UpperLimitBound=90  UpperLimitBoundUnits=deg  UpperLimitStiffness=1e4  UpperLimitStiffnessUnits=N*m/deg  UpperLimitDamping=10  UpperLimitDampingUnits=N*m/(deg/s)  UpperLimitTransitionRegionWidth=0.1  UpperLimitTransitionRegionWidthUnits=deg  PositionTargetSpecify=on  PositionTargetPriority=Low  PositionTargetValue=smiData.RevoluteJoint(11).Rz.Pos  PositionTargetValueUnits=deg  VelocityTargetSpecify=off  VelocityTargetPriority=High  VelocityTargetValue=0  VelocityTargetValueUnits=deg/s
  Revolute11 : sm_lib/Joints/Revolute Joint  SenseConstraintForce=off  SenseConstraintForceX=off  SenseConstraintForceY=off  SenseConstraintForceZ=off  SenseConstraintTorque=off  SenseConstraintTorqueX=off  SenseConstraintTorqueY=off  SenseConstraintTorqueZ=off  SenseTotalForce=off  SenseTotalForceX=off  SenseTotalForceY=off  SenseTotalForceZ=off  SenseTotalTorque=off  SenseTotalTorqueX=off  SenseTotalTorqueY=off  SenseTotalTorqueZ=off  CompositeWrenchDir=FollowerOnBase  CompositeWrenchFrame=BaseFrame  EquilibriumPosition=0  EquilibriumPositionUnits=rad  SpringStiffness=0  SpringStiffnessUnits=N*m/rad  DampingCoefficient=0  DampingCoefficientUnits=N*m/(rad/s)  TorqueActuationMode=NoTorque  MotionActuationMode=ComputedMotion  SensePosition=off  SenseVelocity=off  SenseAcceleration=off  SenseTorqueForce=off  SenseLowerLimitTorqueForce=off  SenseUpperLimitTorqueForce=off  LowerLimitSpecify=off  LowerLimitBound=-90  LowerLimitBoundUnits=deg  LowerLimitStiffness=1e4  LowerLimitStiffnessUnits=N*m/deg  LowerLimitDamping=10  LowerLimitDampingUnits=N*m/(deg/s)  LowerLimitTransitionRegionWidth=0.1  LowerLimitTransitionRegionWidthUnits=deg  UpperLimitSpecify=off  UpperLimitBound=90  UpperLimitBoundUnits=deg  UpperLimitStiffness=1e4  UpperLimitStiffnessUnits=N*m/deg  UpperLimitDamping=10  UpperLimitDampingUnits=N*m/(deg/s)  UpperLimitTransitionRegionWidth=0.1  UpperLimitTransitionRegionWidthUnits=deg  PositionTargetSpecify=on  PositionTargetPriority=Low  PositionTargetValue=smiData.RevoluteJoint(12).Rz.Pos  PositionTargetValueUnits=deg  VelocityTargetSpecify=off  VelocityTargetPriority=High  VelocityTargetValue=0  VelocityTargetValueUnits=deg/s
  Revolute6 : sm_lib/Joints/Revolute Joint  SenseConstraintForce=off  SenseConstraintForceX=off  SenseConstraintForceY=off  SenseConstraintForceZ=off  SenseConstraintTorque=off  SenseConstraintTorqueX=off  SenseConstraintTorqueY=off  SenseConstraintTorqueZ=off  SenseTotalForce=off  SenseTotalForceX=off  SenseTotalForceY=off  SenseTotalForceZ=off  SenseTotalTorque=off  SenseTotalTorqueX=off  SenseTotalTorqueY=off  SenseTotalTorqueZ=off  CompositeWrenchDir=FollowerOnBase  CompositeWrenchFrame=BaseFrame  EquilibriumPosition=0  EquilibriumPositionUnits=rad  SpringStiffness=0  SpringStiffnessUnits=N*m/rad  DampingCoefficient=0  DampingCoefficientUnits=N*m/(rad/s)  TorqueActuationMode=NoTorque  MotionActuationMode=ComputedMotion  SensePosition=off  SenseVelocity=off  SenseAcceleration=off  SenseTorqueForce=off  SenseLowerLimitTorqueForce=off  SenseUpperLimitTorqueForce=off  LowerLimitSpecify=off  LowerLimitBound=-90  LowerLimitBoundUnits=deg  LowerLimitStiffness=1e4  LowerLimitStiffnessUnits=N*m/deg  LowerLimitDamping=10  LowerLimitDampingUnits=N*m/(deg/s)  LowerLimitTransitionRegionWidth=0.1  LowerLimitTransitionRegionWidthUnits=deg  UpperLimitSpecify=off  UpperLimitBound=90  UpperLimitBoundUnits=deg  UpperLimitStiffness=1e4  UpperLimitStiffnessUnits=N*m/deg  UpperLimitDamping=10  UpperLimitDampingUnits=N*m/(deg/s)  UpperLimitTransitionRegionWidth=0.1  UpperLimitTransitionRegionWidthUnits=deg  PositionTargetSpecify=on  PositionTargetPriority=Low  PositionTargetValue=smiData.RevoluteJoint(7).Rz.Pos  PositionTargetValueUnits=deg  VelocityTargetSpecify=off  VelocityTargetPriority=High  VelocityTargetValue=0  VelocityTargetValueUnits=deg/s
  Revolute7 : sm_lib/Joints/Revolute Joint  SenseConstraintForce=off  SenseConstraintForceX=off  SenseConstraintForceY=off  SenseConstraintForceZ=off  SenseConstraintTorque=off  SenseConstraintTorqueX=off  SenseConstraintTorqueY=off  SenseConstraintTorqueZ=off  SenseTotalForce=off  SenseTotalForceX=off  SenseTotalForceY=off  SenseTotalForceZ=off  SenseTotalTorque=off  SenseTotalTorqueX=off  SenseTotalTorqueY=off  SenseTotalTorqueZ=off  CompositeWrenchDir=FollowerOnBase  CompositeWrenchFrame=BaseFrame  EquilibriumPosition=0  EquilibriumPositionUnits=rad  SpringStiffness=0  SpringStiffnessUnits=N*m/rad  DampingCoefficient=0  DampingCoefficientUnits=N*m/(rad/s)  TorqueActuationMode=NoTorque  MotionActuationMode=ComputedMotion  SensePosition=off  SenseVelocity=off  SenseAcceleration=off  SenseTorqueForce=off  SenseLowerLimitTorqueForce=off  SenseUpperLimitTorqueForce=off  LowerLimitSpecify=off  LowerLimitBound=-90  LowerLimitBoundUnits=deg  LowerLimitStiffness=1e4  LowerLimitStiffnessUnits=N*m/deg  LowerLimitDamping=10  LowerLimitDampingUnits=N*m/(deg/s)  LowerLimitTransitionRegionWidth=0.1  LowerLimitTransitionRegionWidthUnits=deg  UpperLimitSpecify=off  UpperLimitBound=90  UpperLimitBoundUnits=deg  UpperLimitStiffness=1e4  UpperLimitStiffnessUnits=N*m/deg  UpperLimitDamping=10  UpperLimitDampingUnits=N*m/(deg/s)  UpperLimitTransitionRegionWidth=0.1  UpperLimitTransitionRegionWidthUnits=deg  PositionTargetSpecify=on  PositionTargetPriority=Low  PositionTargetValue=smiData.RevoluteJoint(8).Rz.Pos  PositionTargetValueUnits=deg  VelocityTargetSpecify=off  VelocityTargetPriority=High  VelocityTargetValue=0  VelocityTargetValueUnits=deg/s
  Revolute8 : sm_lib/Joints/Revolute Joint  SenseConstraintForce=off  SenseConstraintForceX=off  SenseConstraintForceY=off  SenseConstraintForceZ=off  SenseConstraintTorque=off  SenseConstraintTorqueX=off  SenseConstraintTorqueY=off  SenseConstraintTorqueZ=off  SenseTotalForce=off  SenseTotalForceX=off  SenseTotalForceY=off  SenseTotalForceZ=off  SenseTotalTorque=off  SenseTotalTorqueX=off  SenseTotalTorqueY=off  SenseTotalTorqueZ=off  CompositeWrenchDir=FollowerOnBase  CompositeWrenchFrame=BaseFrame  EquilibriumPosition=0  EquilibriumPositionUnits=rad  SpringStiffness=0  SpringStiffnessUnits=N*m/rad  DampingCoefficient=0  DampingCoefficientUnits=N*m/(rad/s)  TorqueActuationMode=NoTorque  MotionActuationMode=ComputedMotion  SensePosition=off  SenseVelocity=off  SenseAcceleration=off  SenseTorqueForce=off  SenseLowerLimitTorqueForce=off  SenseUpperLimitTorqueForce=off  LowerLimitSpecify=off  LowerLimitBound=-90  LowerLimitBoundUnits=deg  LowerLimitStiffness=1e4  LowerLimitStiffnessUnits=N*m/deg  LowerLimitDamping=10  LowerLimitDampingUnits=N*m/(deg/s)  LowerLimitTransitionRegionWidth=0.1  LowerLimitTransitionRegionWidthUnits=deg  UpperLimitSpecify=off  UpperLimitBound=90  UpperLimitBoundUnits=deg  UpperLimitStiffness=1e4  UpperLimitStiffnessUnits=N*m/deg  UpperLimitDamping=10  UpperLimitDampingUnits=N*m/(deg/s)  UpperLimitTransitionRegionWidth=0.1  UpperLimitTransitionRegionWidthUnits=deg  PositionTargetSpecify=on  PositionTargetPriority=Low  PositionTargetValue=smiData.RevoluteJoint(9).Rz.Pos  PositionTargetValueUnits=deg  VelocityTargetSpecify=off  VelocityTargetPriority=High  VelocityTargetValue=0  VelocityTargetValueUnits=deg/s
  Revolute9 : sm_lib/Joints/Revolute Joint  SenseConstraintForce=off  SenseConstraintForceX=off  SenseConstraintForceY=off  SenseConstraintForceZ=off  SenseConstraintTorque=off  SenseConstraintTorqueX=off  SenseConstraintTorqueY=off  SenseConstraintTorqueZ=off  SenseTotalForce=off  SenseTotalForceX=off  SenseTotalForceY=off  SenseTotalForceZ=off  SenseTotalTorque=off  SenseTotalTorqueX=off  SenseTotalTorqueY=off  SenseTotalTorqueZ=off  CompositeWrenchDir=FollowerOnBase  CompositeWrenchFrame=BaseFrame  EquilibriumPosition=0  EquilibriumPositionUnits=rad  SpringStiffness=0  SpringStiffnessUnits=N*m/rad  DampingCoefficient=0  DampingCoefficientUnits=N*m/(rad/s)  TorqueActuationMode=NoTorque  MotionActuationMode=ComputedMotion  SensePosition=off  SenseVelocity=off  SenseAcceleration=off  SenseTorqueForce=off  SenseLowerLimitTorqueForce=off  SenseUpperLimitTorqueForce=off  LowerLimitSpecify=off  LowerLimitBound=-90  LowerLimitBoundUnits=deg  LowerLimitStiffness=1e4  LowerLimitStiffnessUnits=N*m/deg  LowerLimitDamping=10  LowerLimitDampingUnits=N*m/(deg/s)  LowerLimitTransitionRegionWidth=0.1  LowerLimitTransitionRegionWidthUnits=deg  UpperLimitSpecify=off  UpperLimitBound=90  UpperLimitBoundUnits=deg  UpperLimitStiffness=1e4  UpperLimitStiffnessUnits=N*m/deg  UpperLimitDamping=10  UpperLimitDampingUnits=N*m/(deg/s)  UpperLimitTransitionRegionWidth=0.1  UpperLimitTransitionRegionWidthUnits=deg  PositionTargetSpecify=on  PositionTargetPriority=Low  PositionTargetValue=smiData.RevoluteJoint(10).Rz.Pos  PositionTargetValueUnits=deg  VelocityTargetSpecify=off  VelocityTargetPriority=High  VelocityTargetValue=0  VelocityTargetValueUnits=deg/s
  Simulink-PS Converter6 : nesl_utility/Simulink-PS Converter  PhysicalDomain=network_engine_domain  SubClassName=ps_input  LeftPortType=input  RightPortType=output  PseudoPeriodic=off  Frequencies=[]  NoiseDistribution=none  NoiseParameters=[]  Unit=m  AffineConversion=off  FilteringAndDerivatives=filter  SimscapeFilterOrder=2  InputFilterTimeConstant=0.001  UdotUserProvided=0
  Weld Joint : sm_lib/Joints/Weld Joint  SenseConstraintForce=off  SenseConstraintForceX=off  SenseConstraintForceY=off  SenseConstraintForceZ=off  SenseConstraintTorque=off  SenseConstraintTorqueX=off  SenseConstraintTorqueY=off  SenseConstraintTorqueZ=off  SenseTotalForce=off  SenseTotalForceX=off  SenseTotalForceY=off  SenseTotalForceZ=off  SenseTotalTorque=off  SenseTotalTorqueX=off  SenseTotalTorqueY=off  SenseTotalTorqueZ=off  CompositeWrenchDir=FollowerOnBase  CompositeWrenchFrame=BaseFrame
  cap : Subsystem
  main_hand : Subsystem
  scrow : Subsystem
  Conn1 : PMIOPort  Side=Left
  x6 : Outport
  dx6 : Outport  Port=2
  wires:
  q_6/1 -> K6/1
  PS-Simulink Converter5/1 -> x6/1
  K6/1 -> Simulink-PS Converter6/1
  PS-Simulink Converter1/1 -> dx6/1
  connections:
  Simulink-PS Converter6/RConn1 -- Cylindrical Joint/LConn2
  Revolute9/RConn1 -- H2/LConn1
  Revolute Joint2/LConn1 -- cap/RConn1
  Revolute Joint2/RConn1 -- F3/LConn1
  Revolute8/LConn1 -- Hand/RConn2
  PS-Simulink Converter5/LConn1 -- Cylindrical Joint/RConn2
  Revolute11/LConn1 -- F3/RConn1
  Revolute Joint1/LConn1 -- cap/RConn2
  Revolute7/RConn1 -- H1/LConn1
  Revolute1/RConn1 -- scrow/LConn1
  Revolute7/LConn1 -- F1/RConn1
  Revolute6/RConn1 -- H1/LConn2
  Revolute9/LConn1 -- F2/RConn1
  Revolute11/RConn1 -- H3/LConn1
  Revolute Joint/RConn1 -- F1/LConn1
  Revolute10/LConn1 -- Hand/RConn1
  cap/LConn1 -- Weld Joint/RConn1
  Weld Joint/LConn1 -- main_hand/RConn1
  Revolute8/RConn1 -- H2/LConn2
  Revolute Joint1/RConn1 -- F2/LConn1
  Revolute Joint/LConn1 -- cap/RConn3
  Cylindrical Joint/RConn1 -- Hand/LConn1
  Cylindrical Joint/LConn1 -- main_hand/RConn3
  Revolute1/LConn1 -- main_hand/RConn2
  Revolute6/LConn1 -- Hand/RConn3
  Revolute10/RConn1 -- H3/LConn2
  Conn1/RConn1 -- main_hand/LConn1
  PS-Simulink Converter1/LConn1 -- Cylindrical Joint/RConn3

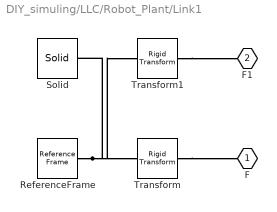
== system DIY_simuling/LLC/Robot_Plant/Link1 ==
  ReferenceFrame : sm_lib/Frames and Transforms/Reference Frame
  Solid : sm_lib/Body Elements/Solid  InertiaType=Custom  Mass=smiData.Solid(2).mass  MassUnits=kg  CenterOfMass=smiData.Solid(2).CoM  CenterOfMassUnits=mm  MomentsOfInertia=smiData.Solid(2).MoI  MomentsOfInertiaUnits=kg*mm^2  ProductsOfInertia=smiData.Solid(2).PoI  ProductsOfInertiaUnits=kg*mm^2  BasedOnType=Density  Density=1000  DensityUnits=kg/m^3  DoExposeReferenceFrame=on  SerializedFrames=<Frames/>  GraphicType=FromGeometry  MarkerShape=Sphere  MarkerSize=10  GraphicVisPropType=SimpleVisualProperties  GraphicDiffuseColor=smiData.Solid(2).color  GraphicSpecularColor=[0.5 0.5 0.5 1.0]  GraphicAmbientColor=[0.15 0.15 0.15 1.0]  GraphicEmissiveColor=[0.0 0.0 0.0 1.0]  GraphicShininess=75  GraphicOpacity=smiData.Solid(2).opacity  GeometryShape=FromFile  RectangleSize=[1 1]  RectangleSizeUnits=m  BrickDimensions=[1 1 1]  BrickDimensionUnits=m  CylinderRadius=1  CylinderRadiusUnits=m  CylinderLength=1  CylinderLengthUnits=m  SphereRadius=1  SphereRadiusUnits=m  EllipsoidRadii=[1 1 1]  EllipsoidRadiiUnits=m  ExtrusionCrossSection=[1 1; -1 1; -1 -1; 1 -1]  ExtrusionCrossSectionUnits=m  ExtrusionLength=1  ExtrusionLengthUnits=m  PolygonNumSides=3  PolygonOuterRadius=1  PolygonOuterRadiusUnits=m  ExtGeomFileType=STEP  ExtGeomFileName=Robot - J1.stp.step_Default_sldprt.STEP  ExtGeomFileUnits=m  RevolutionCrossSection=[1 1; 1 -1; 2 -1; 2 1]  RevolutionCrossSectionUnits=m  RevolutionExtent=Full  RevolutionAngle=180  RevolutionAngleUnits=deg
  Transform : sm_lib/Frames and Transforms/Rigid Transform  TranslationMethod=Cartesian  TranslationStandardOffset=0  TranslationLengthUnit=mm  TranslationStandardAxis=+Z  TranslationCartesianOffset=smiData.RigidTransform(10).translation  TranslationROffset=0  TranslationROffsetUnits=m  TranslationZOffset=0  TranslationZOffsetUnits=m  TranslationThetaOffset=0  TranslationThetaOffsetUnits=deg  RotationMethod=ArbitraryAxis  RotationAngleUnits=rad  RotationStandardAxis=+Z  RotationAngle=smiData.RigidTransform(10).angle  RotationArbitraryAxis=smiData.RigidTransform(10).axis  FollAlignAxisA=+X  BaseAlignAxisA=+Y  FollAlignAxisB=+Y  BaseAlignAxisB=+Z  RotationSequenceAxes=FollowerAxes  RotationSequence=XYX  RotationSequenceAngles=[0 0 0]  RotationSequenceAnglesUnits=deg  RotationMatrix=[1 0 0; 0 1 0; 0 0 1]
  Transform1 : sm_lib/Frames and Transforms/Rigid Transform  TranslationMethod=Cartesian  TranslationStandardOffset=0  TranslationLengthUnit=mm  TranslationStandardAxis=+Z  TranslationCartesianOffset=smiData.RigidTransform(11).translation  TranslationROffset=0  TranslationROffsetUnits=m  TranslationZOffset=0  TranslationZOffsetUnits=m  TranslationThetaOffset=0  TranslationThetaOffsetUnits=deg  RotationMethod=ArbitraryAxis  RotationAngleUnits=rad  RotationStandardAxis=+Z  RotationAngle=smiData.RigidTransform(11).angle  RotationArbitraryAxis=smiData.RigidTransform(11).axis  FollAlignAxisA=+X  BaseAlignAxisA=+Y  FollAlignAxisB=+Y  BaseAlignAxisB=+Z  RotationSequenceAxes=FollowerAxes  RotationSequence=XYX  RotationSequenceAngles=[0 0 0]  RotationSequenceAnglesUnits=deg  RotationMatrix=[1 0 0; 0 1 0; 0 0 1]
  F : PMIOPort  Side=Left
  F1 : PMIOPort  Port=2  Side=Right
  connections:
  Solid/RConn1 -- ReferenceFrame/RConn1 -- Transform/LConn1 -- Transform1/LConn1
  Transform/RConn1 -- F/RConn1
  Transform1/RConn1 -- F1/RConn1
